simulink model "tg9"  (R2022a)
settings: Solver=ode15s  StartTime=0.0  StopTime=10  MaxStep=0.01  RelTol=1e-3
InitFcn:
  | mecha_param2
  | control_param0
values from neighbouring files (symbols this model uses):
  b0 = 0    [sim_IMMC.m]
  b1 = 1    [sim_IMMC.m]
  back0 = 0    [sim_IMMC.m]
  back1 = 0    [sim_IMMC.m]
  boff = 0    [sim_IMMC.m]
  bon = 0    [sim_IMMC.m]
  c = 0.05    [mecha_param2.m]
  c_jointstop = 0.3 / (pi/180)    (= 17.1887338539)    [mecha_param2.m]
  calctalus = sqrt((L_foot - (DJ1x_foot))^2 + (H_foot-r_cs)^2)    [mecha_param2.m]
  calctoes = sqrt((H_foot-r_cs)^2 + (DJ1x_foot)^2)    [mecha_param2.m]
  corrD = 0.001    [control_param0.m]
  DG_HAT = 0.35    [mecha_param2.m]
  DG_thigh = 0.28    [mecha_param2.m]
  DJ1x_foot = 0.16-r_cs    (= 0.135)    [mecha_param2.m]
  eref = 0.04    [mecha_param2.m]
  FmaxBFSH = 350    [mecha_param2.m]
  FmaxGAS = 1500    [mecha_param2.m]
  FmaxGLU = 1500    [mecha_param2.m]
  FmaxHAM = 3000    [mecha_param2.m]
  FmaxHFL = 2000    [mecha_param2.m]
  FmaxRF = 1200    [mecha_param2.m]
  FmaxSOL = 4000    [mecha_param2.m]
  FmaxTA = 800    [mecha_param2.m]
  FmaxVAS = 6000    [mecha_param2.m]
  g = 9.81    [mecha_param2.m]
  g0 = 0    [sim_IMMC.m]
  g1 = 0    [sim_IMMC.m]
  H_foot = 0.08    [mecha_param2.m]
  In_HAT = 3    [mecha_param2.m]
  In_shank = 0.05    [mecha_param2.m]
  In_thigh = 0.15    [mecha_param2.m]
  K = 5    [mecha_param2.m]
  knee_thigh = [0 0 -(L_thigh/2)]    [mecha_param2.m]
  Kpress = m_HAT * g / DeltaThRef    (= 104967)    [mecha_param2.m]
  L_foot = 0.2    [mecha_param2.m]
  L_HAT = 0.8    [mecha_param2.m]
  L_shank = 0.46    [mecha_param2.m]
  L_thigh = 0.46    [mecha_param2.m]
  LoHAM = table2array(mt('LoHAM', 1))    [control_param0.m]
  LoHFL = table2array(mt('LoHFL', 1))    [control_param0.m]
  longD = longD - corrD    (= 0.019)    [control_param0.m]
  loptBFSH = 0.12    [mecha_param2.m]
  loptGAS = 0.05    [mecha_param2.m]
  loptGLU = 0.11    [mecha_param2.m]
  loptHAM = 0.10    (= 0.1)    [mecha_param2.m]
  loptHFL = 0.11    [mecha_param2.m]
  loptRF = 0.08    [mecha_param2.m]
  loptSOL = 0.04    [mecha_param2.m]
  loptTA = 0.06    [mecha_param2.m]
  loptVAS = 0.08    [mecha_param2.m]
  LoTA = table2array(mt('LoTA', 1))    [control_param0.m]
  lslackBFSH = 0.10    (= 0.1)    [mecha_param2.m]
  lslackGAS = 0.40    (= 0.4)    [mecha_param2.m]
  lslackGLU = 0.13    [mecha_param2.m]
  lslackHAM = 0.31    [mecha_param2.m]
  lslackHFL = 0.10    (= 0.1)    [mecha_param2.m]
  lslackRF = 0.35    [mecha_param2.m]
  lslackSOL = 0.26    [mecha_param2.m]
  lslackTA = 0.24    [mecha_param2.m]
  lslackVAS = 0.23    [mecha_param2.m]
  m_HAT = 53.5    [mecha_param2.m]
  m_shank = 3.5    [mecha_param2.m]
  m_thigh = 8.5    [mecha_param2.m]
  midD = midD - corrD    (= 0.009)    [control_param0.m]
  N = 1.5    [mecha_param2.m]
  nonoff = 0    [control_param0.m]
  phi_a_low = (70) * (pi / 180)    (= 1.2217304764)    [mecha_param2.m]
  phi_a_up = (130) * (pi / 180)    (= 2.26892802759)    [mecha_param2.m]
  phi_dl = 180    [mecha_param2.m]
  phi_h = 230 * (pi / 180)    (= 4.01425727959)    [mecha_param2.m]
  phi_k = 175 * (pi / 180)    (= 3.05432619099)    [mecha_param2.m]
  phictoes = asind((DJ1y_foot-r_cs)/calctoes)    [mecha_param2.m]
  phimaxGASa = 100*pi/180    (= 1.74532925199)    [mecha_param2.m]
  phimaxGASk = 140*pi/180    (= 2.44346095279)    [mecha_param2.m]
  phimaxRFk = 165*pi/180    (= 2.87979326579)    [mecha_param2.m]
  phimaxSOL = 100*pi/180    (= 1.74532925199)    [mecha_param2.m]
  phimaxTA = 80*pi/180    (= 1.3962634016)    [mecha_param2.m]
  phimaxVAS = 165*pi/180    (= 2.87979326579)    [mecha_param2.m]
  phirefBFSH = 160*pi/180    (= 2.79252680319)    [mecha_param2.m]
  phirefGASa = 80*pi/180    (= 1.3962634016)    [mecha_param2.m]
  phirefGASk = 165*pi/180    (= 2.87979326579)    [mecha_param2.m]
  phirefGLU = 120*pi/180    (= 2.09439510239)    [mecha_param2.m]
  phirefHAMh = 150*pi/180    (= 2.61799387799)    [mecha_param2.m]
  phirefHAMk = 180*pi/180    (= 3.14159265359)    [mecha_param2.m]
  phirefHFL = 160*pi/180    (= 2.79252680319)    [mecha_param2.m]
  phirefRFh = 170*pi/180    (= 2.96705972839)    [mecha_param2.m]
  phirefRFk = 125*pi/180    (= 2.18166156499)    [mecha_param2.m]
  phirefSOL = 90*pi/180    (= 1.57079632679)    [mecha_param2.m]
  phirefTA = 110*pi/180    (= 1.91986217719)    [mecha_param2.m]
  phirefVAS = 120*pi/180    (= 2.09439510239)    [mecha_param2.m]
  phiScaleGASa = acos(rGASamin/rGASamax)/(phiminGASa-phimaxGASa)    [mecha_param2.m]
  phiScaleGASk = acos(rGASkmin/rGASkmax)/(phiminGASk-phimaxGASk)    [mecha_param2.m]
  phiScaleRFk = acos(rRFkmin/rRFkmax)/(phiminRFk-phimaxRFk)    [mecha_param2.m]
  phiScaleSOL = acos(rSOLmin/rSOLmax)/(phiminSOL-phimaxSOL)    [mecha_param2.m]
  phiScaleTA = acos(rTAmin/rTAmax)/(phiminTA-phimaxTA)    [mecha_param2.m]
  phiScaleVAS = acos(rVASmin/rVASmax)/(phiminVAS-phimaxVAS)    [mecha_param2.m]
  r1 = 0    [sim_IMMC.m]
  r_cs = 0.025    [mecha_param2.m]
  rBFSH = 0.04    [mecha_param2.m]
  rGASamax = 0.06    [mecha_param2.m]
  rGASkmax = 0.05    [mecha_param2.m]
  rGLU = 0.08    [mecha_param2.m]
  rHAMh = 0.08    [mecha_param2.m]
  rHAMk = 0.05    [mecha_param2.m]
  rHFL = 0.08    [mecha_param2.m]
  rhoBFSH = 0.7    [mecha_param2.m]
  rhoGASa = 0.7    [mecha_param2.m]
  rhoGASk = 0.7    [mecha_param2.m]
  rhoGLU = 0.5    [mecha_param2.m]
  rhoHAMh = 0.5    [mecha_param2.m]
  rhoHAMk = 0.5    [mecha_param2.m]
  rhoHFL = 0.5    [mecha_param2.m]
  rhoRFh = 0.3    [mecha_param2.m]
  rhoRFk = 0.5    [mecha_param2.m]
  rhoSOL = 0.5    [mecha_param2.m]
  rhoTA = 0.7    [mecha_param2.m]
  rhoVAS = 0.6    [mecha_param2.m]
  rRFh = 0.08    [mecha_param2.m]
  rRFkmax = 0.06    [mecha_param2.m]
  rSOLmax = 0.06    [mecha_param2.m]
  ... (+25 more)
undefined symbols (not defined in the file or in its folder): beta11, beta12, beta13, beta14, beta15, beta16, beta21, beta22, beta23, beta24, beta25, beta26, beta31, beta32, beta33, beta34, beta35, beta36, beta41, beta42, beta43, beta44, beta45, beta46, beta51, beta52, beta53, beta54, beta55, beta56, betab1, betab2, betab3, betab4, betab5, betab6, betap11, betap12, betap13, betap14, betap15, betap16, betap21, betap22, betap23, betap24, betap25, betap26, betap31, betap32, betap33, betap34, betap35, betap36, betap41, betap42, betap43, betap44, betap45, betap46 ... (+102)
libraries: sm_lib x89, simulink x72, nesl_utility x58, simulink_extras x18
(part 4 of 12)

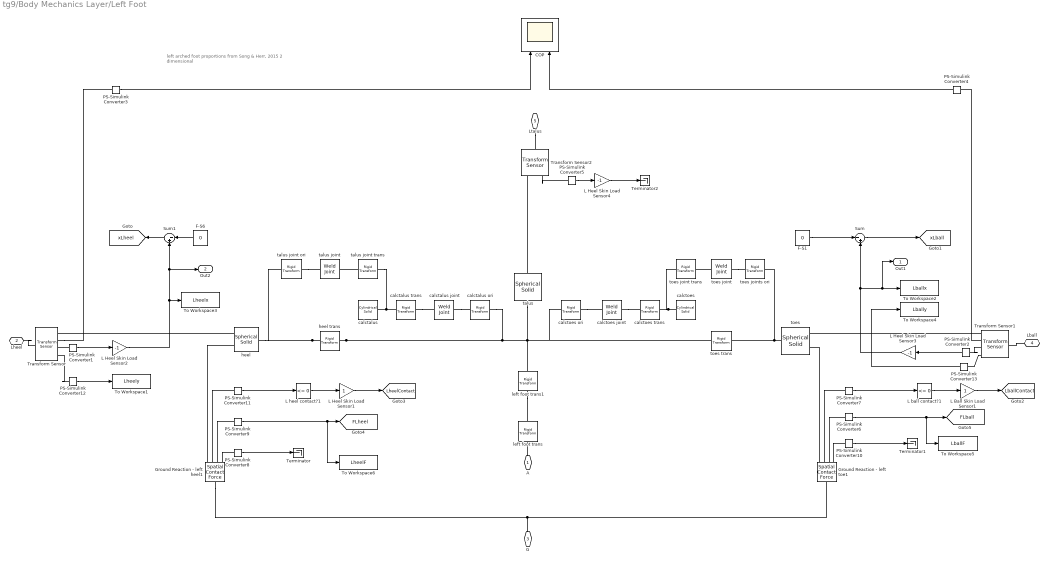
== system tg9/Body Mechanics Layer/Left Foot ==
  note: left arched foot
      | proportions from Song & Herr, 2015
      | 2 dimensional
  COP : Scope  NumInputPorts=2
  F-S1 : Constant  Value=0  OutDataTypeStr=Inherit: Inherit via back propagation
  F-S6 : Constant  Value=0  OutDataTypeStr=Inherit: Inherit via back propagation
  Ground Reaction - left heel1 : sm_lib/Forces and Torques/Spatial Contact Force  SenseContactBaseRotation=off  SenseContactBaseTranslation=off  CoefficientOfDynamicFriction=mu_static  CoefficientOfStaticFriction=mu_dynamic  NormalDamping=damp  NormalDampingUnits=N/(m/s)  SenseContactSignal=off  NormalStiffness=stiff  NormalStiffnessUnits=N/m  FrictionalCriticalVelocity=vLimit  FrictionalCriticalVelocityUnits=m/s  ZeroCrossDetectContactStartAndEnd=on  SenseContactFollowerRotation=off  SenseContactFollowerTranslation=off  FrictionType=SmoothStickSlip  SenseFrictionalForceMagnitude=on  SenseNormalForceMagnitude=on  NormalForceType=SmoothSpringDamper  SenseNormalVelocity=off  SenseSeparationDistance=on  SenseTangentialVelocity=off  NormalTransitionRegionWidth=trw  NormalTransitionRegionWidthUnits=m
  Ground Reaction - left toe1 : sm_lib/Forces and Torques/Spatial Contact Force  SenseContactBaseRotation=off  SenseContactBaseTranslation=off  CoefficientOfDynamicFriction=mu_static  CoefficientOfStaticFriction=mu_dynamic  NormalDamping=damp  NormalDampingUnits=N/(m/s)  SenseContactSignal=off  NormalStiffness=stiff  NormalStiffnessUnits=N/m  FrictionalCriticalVelocity=vLimit  FrictionalCriticalVelocityUnits=m/s  ZeroCrossDetectContactStartAndEnd=on  SenseContactFollowerRotation=off  SenseContactFollowerTranslation=off  FrictionType=SmoothStickSlip  SenseFrictionalForceMagnitude=on  SenseNormalForceMagnitude=on  NormalForceType=SmoothSpringDamper  SenseNormalVelocity=off  SenseSeparationDistance=on  SenseTangentialVelocity=off  NormalTransitionRegionWidth=trw  NormalTransitionRegionWidthUnits=m
  L Ball Skin Load Sensor1 : Gain
  L Heel Skin Load Sensor1 : Gain
  L Heel Skin Load Sensor2 : Gain  Gain=-1
  L Heel Skin Load Sensor3 : Gain  Gain=-1
  L Heel Skin Load Sensor4 : Gain  Gain=-1
  L ball contact?1 : simulink/Logic and Bit Operations/Compare To Zero  relop=<=  OutDataTypeStr=boolean
  L heel contact?1 : simulink/Logic and Bit Operations/Compare To Zero  relop=<=  OutDataTypeStr=boolean
  PS-Simulink Converter{1..13} (13 alike) : nesl_utility/PS-Simulink Converter  PhysicalDomain=network_engine_domain  SubClassName=ps_output  LeftPortType=input  RightPortType=output  PseudoPeriodic=off  Frequencies=[]  VectorFormat=1-D array  Unit=inherit  AffineConversion=off
      settings: SourceProductBaseCode=SS,PW,VE
  Sum : Sum  Inputs=|-+
  Sum1 : Sum  Inputs=|-+
  Terminator : Terminator
  Terminator1 : Terminator
  Terminator2 : Terminator
  To Workspace1 : ToWorkspace  VariableName=Lheely  SampleTime=-1
  To Workspace2 : ToWorkspace  VariableName=Lballx  SampleTime=-1
  To Workspace3 : ToWorkspace  VariableName=Lheelx  SampleTime=-1
  To Workspace4 : ToWorkspace  VariableName=Lbally  SampleTime=-1
  To Workspace5 : ToWorkspace  VariableName=LballF  SampleTime=-1
  To Workspace6 : ToWorkspace  VariableName=LheelF  SampleTime=-1
  Transform Sensor : sm_lib/Frames and Transforms/Transform Sensor  MeasurementFrame=World  SenseAngle=off  SenseAxis=off  SenseAngle1=off  SenseAngle2=off  SenseAngle3=off  SenseQ=off  SenseR=off  SenseOmegaX=off  SenseOmegaY=off  SenseOmegaZ=off  SenseOmega1=off  SenseOmega2=off  SenseOmega3=off  SenseQDot=off  SenseRDot=off  SenseAlphaX=off  SenseAlphaY=off  SenseAlphaZ=off  SenseAlpha1=off  SenseAlpha2=off  SenseAlpha3=off  SenseQDDot=off  SenseRDDot=off  SenseX=on  SenseY=on  SenseZ=on  SenseRad=off  SenseAzim=off  SenseDist=off  SenseInc=off  SenseXDot=off  SenseYDot=off  SenseZDot=off  SenseRadDot=off  SenseAzimDot=off  SenseDistDot=off  SenseIncDot=off  SenseXDDot=off  SenseYDDot=off  SenseZDDot=off  SenseRadDDot=off  SenseAzimDDot=off  SenseDistDDot=off  SenseIncDDot=off
  Transform Sensor1 : sm_lib/Frames and Transforms/Transform Sensor  MeasurementFrame=World  SenseAngle=off  SenseAxis=off  SenseAngle1=off  SenseAngle2=off  SenseAngle3=off  SenseQ=off  SenseR=off  SenseOmegaX=off  SenseOmegaY=off  SenseOmegaZ=off  SenseOmega1=off  SenseOmega2=off  SenseOmega3=off  SenseQDot=off  SenseRDot=off  SenseAlphaX=off  SenseAlphaY=off  SenseAlphaZ=off  SenseAlpha1=off  SenseAlpha2=off  SenseAlpha3=off  SenseQDDot=off  SenseRDDot=off  SenseX=on  SenseY=on  SenseZ=on  SenseRad=off  SenseAzim=off  SenseDist=off  SenseInc=off  SenseXDot=off  SenseYDot=off  SenseZDot=off  SenseRadDot=off  SenseAzimDot=off  SenseDistDot=off  SenseIncDot=off  SenseXDDot=off  SenseYDDot=off  SenseZDDot=off  SenseRadDDot=off  SenseAzimDDot=off  SenseDistDDot=off  SenseIncDDot=off
  Transform Sensor2 : sm_lib/Frames and Transforms/Transform Sensor  MeasurementFrame=World  SenseAngle=off  SenseAxis=off  SenseAngle1=off  SenseAngle2=off  SenseAngle3=off  SenseQ=off  SenseR=off  SenseOmegaX=off  SenseOmegaY=off  SenseOmegaZ=off  SenseOmega1=off  SenseOmega2=off  SenseOmega3=off  SenseQDot=off  SenseRDot=off  SenseAlphaX=off  SenseAlphaY=off  SenseAlphaZ=off  SenseAlpha1=off  SenseAlpha2=off  SenseAlpha3=off  SenseQDDot=off  SenseRDDot=off  SenseX=off  SenseY=on  SenseZ=off  SenseRad=off  SenseAzim=off  SenseDist=off  SenseInc=off  SenseXDot=off  SenseYDot=off  SenseZDot=off  SenseRadDot=off  SenseAzimDot=off  SenseDistDot=off  SenseIncDot=off  SenseXDDot=off  SenseYDDot=off  SenseZDDot=off  SenseRadDDot=off  SenseAzimDDot=off  SenseDistDDot=off  SenseIncDDot=off
  calctalus : sm_lib/Body Elements/Cylindrical Solid  GraphicAmbientColor=[0.15 0.15 0.15 1.0]  BasedOnType=Mass  CenterOfMass=[0 0 0]  CenterOfMassUnits=m  GraphicDiffuseColor=[0.5 0.5 0.5]  CylinderLength=calctalus  CylinderLengthUnits=m  CylinderRadius=0.02  CylinderRadiusUnits=m  Density=1000  DensityUnits=kg/m^3  DoExposeReferenceFrame=on  GraphicEmissiveColor=[0.0 0.0 0.0 1.0]  ExportEntireGeometry=off  SerializedFrames=<Frames/>  MarkerShape=Sphere  MarkerSize=10  GraphicType=FromGeometry  InertiaType=CalculateFromGeometry  Mass=0  MassUnits=kg  MomentsOfInertia=[1 1 1]  MomentsOfInertiaUnits=kg*m^2  GraphicOpacity=1.0  ProductsOfInertia=[0 0 0]  ProductsOfInertiaUnits=kg*m^2  GraphicShininess=75  GraphicSpecularColor=[0.5 0.5 0.5 1.0]  GraphicVisPropType=SimpleVisualProperties
  calctalus joint : sm_lib/Joints/Weld Joint  JointMode=Normal  SenseConstraintForce=off  SenseConstraintForceX=off  SenseConstraintForceY=off  SenseConstraintForceZ=off  SenseConstraintTorque=off  SenseConstraintTorqueX=off  SenseConstraintTorqueY=off  SenseConstraintTorqueZ=off  SenseTotalForce=off  SenseTotalForceX=off  SenseTotalForceY=off  SenseTotalForceZ=off  SenseTotalTorque=off  SenseTotalTorqueX=off  SenseTotalTorqueY=off  SenseTotalTorqueZ=off  CompositeWrenchDir=FollowerOnBase  CompositeWrenchFrame=BaseFrame
  calctalus ori : sm_lib/Frames and Transforms/Rigid Transform  TranslationMethod=None  TranslationStandardOffset=0  TranslationLengthUnit=m  TranslationStandardAxis=+Z  TranslationCartesianOffset=[0 0 -(calctoes/2)]  TranslationROffset=0  TranslationROffsetUnits=m  TranslationZOffset=0  TranslationZOffsetUnits=m  TranslationThetaOffset=0  TranslationThetaOffsetUnits=deg  RotationMethod=StandardAxis  RotationAngleUnits=deg  RotationStandardAxis=+Y  RotationAngle=phictalus  RotationArbitraryAxis=[0 0 1]  FollAlignAxisA=+X  BaseAlignAxisA=+Y  FollAlignAxisB=+Y  BaseAlignAxisB=+Z  RotationSequenceAxes=FollowerAxes  RotationSequence=XYX  RotationSequenceAngles=[0 0 0]  RotationSequenceAnglesUnits=deg  RotationMatrix=[1 0 0; 0 1 0; 0 0 1]
  calctalus trans : sm_lib/Frames and Transforms/Rigid Transform  TranslationMethod=Cartesian  TranslationStandardOffset=0  TranslationLengthUnit=m  TranslationStandardAxis=+Z  TranslationCartesianOffset=[0 0 -(calctalus/2)]  TranslationROffset=0  TranslationROffsetUnits=m  TranslationZOffset=0  TranslationZOffsetUnits=m  TranslationThetaOffset=0  TranslationThetaOffsetUnits=deg  RotationMethod=None  RotationAngleUnits=deg  RotationStandardAxis=+Y  RotationAngle=phictalus  RotationArbitraryAxis=[0 0 1]  FollAlignAxisA=+X  BaseAlignAxisA=+Y  FollAlignAxisB=+Y  BaseAlignAxisB=+Z  RotationSequenceAxes=FollowerAxes  RotationSequence=XYX  RotationSequenceAngles=[0 0 0]  RotationSequenceAnglesUnits=deg  RotationMatrix=[1 0 0; 0 1 0; 0 0 1]
  calctoes : sm_lib/Body Elements/Cylindrical Solid  GraphicAmbientColor=[0.15 0.15 0.15 1.0]  BasedOnType=Mass  CenterOfMass=[0 0 0]  CenterOfMassUnits=m  GraphicDiffuseColor=[0.5 0.5 0.5]  CylinderLength=calctoes  CylinderLengthUnits=m  CylinderRadius=0.02  CylinderRadiusUnits=m  Density=1000  DensityUnits=kg/m^3  DoExposeReferenceFrame=on  GraphicEmissiveColor=[0.0 0.0 0.0 1.0]  ExportEntireGeometry=off  SerializedFrames=<Frames/>  MarkerShape=Sphere  MarkerSize=10  GraphicType=FromGeometry  InertiaType=CalculateFromGeometry  Mass=0  MassUnits=kg  MomentsOfInertia=[1 1 1]  MomentsOfInertiaUnits=kg*m^2  GraphicOpacity=1.0  ProductsOfInertia=[0 0 0]  ProductsOfInertiaUnits=kg*m^2  GraphicShininess=75  GraphicSpecularColor=[0.5 0.5 0.5 1.0]  GraphicVisPropType=SimpleVisualProperties
  calctoes joint : sm_lib/Joints/Weld Joint  JointMode=Normal  SenseConstraintForce=off  SenseConstraintForceX=off  SenseConstraintForceY=off  SenseConstraintForceZ=off  SenseConstraintTorque=off  SenseConstraintTorqueX=off  SenseConstraintTorqueY=off  SenseConstraintTorqueZ=off  SenseTotalForce=off  SenseTotalForceX=off  SenseTotalForceY=off  SenseTotalForceZ=off  SenseTotalTorque=off  SenseTotalTorqueX=off  SenseTotalTorqueY=off  SenseTotalTorqueZ=off  CompositeWrenchDir=FollowerOnBase  CompositeWrenchFrame=BaseFrame
  calctoes ori : sm_lib/Frames and Transforms/Rigid Transform  TranslationMethod=None  TranslationStandardOffset=0  TranslationLengthUnit=m  TranslationStandardAxis=+Z  TranslationCartesianOffset=[0 0 -(calctoes/2)]  TranslationROffset=0  TranslationROffsetUnits=m  TranslationZOffset=0  TranslationZOffsetUnits=m  TranslationThetaOffset=0  TranslationThetaOffsetUnits=deg  RotationMethod=StandardAxis  RotationAngleUnits=deg  RotationStandardAxis=-Y  RotationAngle=90-phictoes  RotationArbitraryAxis=[0 0 1]  FollAlignAxisA=+X  BaseAlignAxisA=+Y  FollAlignAxisB=+Y  BaseAlignAxisB=+Z  RotationSequenceAxes=FollowerAxes  RotationSequence=XYX  RotationSequenceAngles=[0 0 0]  RotationSequenceAnglesUnits=deg  RotationMatrix=[1 0 0; 0 1 0; 0 0 1]
  calctoes trans : sm_lib/Frames and Transforms/Rigid Transform  TranslationMethod=Cartesian  TranslationStandardOffset=0  TranslationLengthUnit=m  TranslationStandardAxis=+Z  TranslationCartesianOffset=[0 0 -(calctoes/2)]  TranslationROffset=0  TranslationROffsetUnits=m  TranslationZOffset=0  TranslationZOffsetUnits=m  TranslationThetaOffset=0  TranslationThetaOffsetUnits=deg  RotationMethod=None  RotationAngleUnits=deg  RotationStandardAxis=-Y  RotationAngle=90-phictoes  RotationArbitraryAxis=[0 0 1]  FollAlignAxisA=+X  BaseAlignAxisA=+Y  FollAlignAxisB=+Y  BaseAlignAxisB=+Z  RotationSequenceAxes=FollowerAxes  RotationSequence=XYX  RotationSequenceAngles=[0 0 0]  RotationSequenceAnglesUnits=deg  RotationMatrix=[1 0 0; 0 1 0; 0 0 1]
  heel : sm_lib/Body Elements/Spherical Solid  GraphicAmbientColor=[0.15 0.15 0.15 1.0]  BasedOnType=Mass  CenterOfMass=[0 0 0]  CenterOfMassUnits=m  GraphicDiffuseColor=[1.0 0.0 0.2]  Density=1000  DensityUnits=kg/m^3  DoExposeReferenceFrame=on  GraphicEmissiveColor=[0.0 0.0 0.0 1.0]  ExportEntireGeometry=on  SerializedExposedGeometries=<ExposedGeometries/>  SerializedFrames=<Frames><Frame><Id>Frame1</Id><Value><Name>COM</Name><Origin><Source>CenterOfMassFrame</Source><FeatureName></FeatureName></Origin><PrimaryAxis><DefinedDirection>+Z</DefinedDirection><Source>ReferenceFrame</Source><SourceDirection>+Z</SourceDirection><FeatureName></FeatureName></PrimaryAxis><SecondaryAxis><DefinedDirection>+X</DefinedDirection><Source>ReferenceFrame</Source><SourceDirection>+X</SourceDirection><FeatureName></FeatureName></SecondaryAxis></Value></Frame></Frames>  MarkerShape=Sphere  MarkerSize=10  GraphicType=FromGeometry  InertiaType=CalculateFromGeometry  Mass=0  MassUnits=kg  MomentsOfInertia=[1 1 1]  MomentsOfInertiaUnits=kg*m^2  GraphicOpacity=1.0  ProductsOfInertia=[0 0 0]  ProductsOfInertiaUnits=kg*m^2  GraphicShininess=75  GraphicSpecularColor=[0.5 0.5 0.5 1.0]  SphereRadius=r_cs  SphereRadiusUnits=m  GraphicVisPropType=SimpleVisualProperties
  heel trans : sm_lib/Frames and Transforms/Rigid Transform  TranslationMethod=Cartesian  TranslationStandardOffset=0  TranslationLengthUnit=m  TranslationStandardAxis=+Z  TranslationCartesianOffset=[(DJ1x_foot - L_foot) 0 (r_cs-H_foot)]  TranslationROffset=0  TranslationROffsetUnits=m  TranslationZOffset=0  TranslationZOffsetUnits=m  TranslationThetaOffset=0  TranslationThetaOffsetUnits=deg  RotationMethod=None  RotationAngleUnits=deg  RotationStandardAxis=+Y  RotationAngle=phictalus  RotationArbitraryAxis=[0 0 1]  FollAlignAxisA=+X  BaseAlignAxisA=+Y  FollAlignAxisB=+Y  BaseAlignAxisB=+Z  RotationSequenceAxes=FollowerAxes  RotationSequence=XYX  RotationSequenceAngles=[0 0 0]  RotationSequenceAnglesUnits=deg  RotationMatrix=[1 0 0; 0 1 0; 0 0 1]
  left foot trans : sm_lib/Frames and Transforms/Rigid Transform  TranslationMethod=None  TranslationStandardOffset=0  TranslationLengthUnit=m  TranslationStandardAxis=+Z  TranslationCartesianOffset=[]  TranslationROffset=0  TranslationROffsetUnits=m  TranslationZOffset=0  TranslationZOffsetUnits=m  TranslationThetaOffset=0  TranslationThetaOffsetUnits=deg  RotationMethod=StandardAxis  RotationAngleUnits=deg  RotationStandardAxis=+Y  RotationAngle=90  RotationArbitraryAxis=[0 0 1]  FollAlignAxisA=+X  BaseAlignAxisA=+Y  FollAlignAxisB=+Y  BaseAlignAxisB=+Z  RotationSequenceAxes=FollowerAxes  RotationSequence=XYX  RotationSequenceAngles=[0 0 0]  RotationSequenceAnglesUnits=deg  RotationMatrix=[1 0 0; 0 1 0; 0 0 1]
  left foot trans1 : sm_lib/Frames and Transforms/Rigid Transform  TranslationMethod=None  TranslationStandardOffset=0  TranslationLengthUnit=m  TranslationStandardAxis=+Z  TranslationCartesianOffset=[]  TranslationROffset=0  TranslationROffsetUnits=m  TranslationZOffset=0  TranslationZOffsetUnits=m  TranslationThetaOffset=0  TranslationThetaOffsetUnits=deg  RotationMethod=StandardAxis  RotationAngleUnits=deg  RotationStandardAxis=-Z  RotationAngle=90  RotationArbitraryAxis=[0 0 1]  FollAlignAxisA=+X  BaseAlignAxisA=+Y  FollAlignAxisB=+Y  BaseAlignAxisB=+Z  RotationSequenceAxes=FollowerAxes  RotationSequence=XYX  RotationSequenceAngles=[0 0 0]  RotationSequenceAnglesUnits=deg  RotationMatrix=[1 0 0; 0 1 0; 0 0 1]
  talus : sm_lib/Body Elements/Spherical Solid  GraphicAmbientColor=[0.15 0.15 0.15 1.0]  BasedOnType=Density  CenterOfMass=cm_foot  CenterOfMassUnits=m  GraphicDiffuseColor=[0.6 1.0 1.0]  Density=1000  DensityUnits=kg/m^3  DoExposeReferenceFrame=on  GraphicEmissiveColor=[0.0 0.0 0.0 1.0]  ExportEntireGeometry=off  SerializedExposedGeometries=<ExposedGeometries/>  SerializedFrames=<Frames><Frame><Id>Frame1</Id><Value><Name>COM</Name><Origin><Source>ReferenceFrame</Source><FeatureName></FeatureName></Origin><PrimaryAxis><DefinedDirection>+Z</DefinedDirection><Source>ReferenceFrame</Source><SourceDirection>+Z</SourceDirection><FeatureName></FeatureName></PrimaryAxis><SecondaryAxis><DefinedDirection>+X</DefinedDirection><Source>ReferenceFrame</Source><SourceDirection>+X</SourceDirection><FeatureName></FeatureName></SecondaryAxis></Value></Frame></Frames>  MarkerShape=Sphere  MarkerSize=10  GraphicType=FromGeometry  InertiaType=Custom  Mass=1.25  MassUnits=kg  MomentsOfInertia=[0 0.005 0]  MomentsOfInertiaUnits=kg*m^2  GraphicOpacity=1.0  ProductsOfInertia=[0 0 0]  ProductsOfInertiaUnits=kg*m^2  GraphicShininess=75  GraphicSpecularColor=[0.5 0.5 0.5 1.0]  SphereRadius=r_foot  SphereRadiusUnits=m  GraphicVisPropType=SimpleVisualProperties
  talus joint : sm_lib/Joints/Weld Joint  JointMode=Normal  SenseConstraintForce=off  SenseConstraintForceX=off  SenseConstraintForceY=off  SenseConstraintForceZ=off  SenseConstraintTorque=off  SenseConstraintTorqueX=off  SenseConstraintTorqueY=off  SenseConstraintTorqueZ=off  SenseTotalForce=off  SenseTotalForceX=off  SenseTotalForceY=off  SenseTotalForceZ=off  SenseTotalTorque=off  SenseTotalTorqueX=off  SenseTotalTorqueY=off  SenseTotalTorqueZ=off  CompositeWrenchDir=FollowerOnBase  CompositeWrenchFrame=BaseFrame
  talus joint ori : sm_lib/Frames and Transforms/Rigid Transform  TranslationMethod=None  TranslationStandardOffset=0  TranslationLengthUnit=m  TranslationStandardAxis=+Z  TranslationCartesianOffset=[0 0 -(calctoes/2)]  TranslationROffset=0  TranslationROffsetUnits=m  TranslationZOffset=0  TranslationZOffsetUnits=m  TranslationThetaOffset=0  TranslationThetaOffsetUnits=deg  RotationMethod=StandardAxis  RotationAngleUnits=deg  RotationStandardAxis=-Y  RotationAngle=phictalus  RotationArbitraryAxis=[0 0 1]  FollAlignAxisA=+X  BaseAlignAxisA=+Y  FollAlignAxisB=+Y  BaseAlignAxisB=+Z  RotationSequenceAxes=FollowerAxes  RotationSequence=XYX  RotationSequenceAngles=[0 0 0]  RotationSequenceAnglesUnits=deg  RotationMatrix=[1 0 0; 0 1 0; 0 0 1]
  talus joint trans : sm_lib/Frames and Transforms/Rigid Transform  TranslationMethod=Cartesian  TranslationStandardOffset=0  TranslationLengthUnit=m  TranslationStandardAxis=+Z  TranslationCartesianOffset=[0 0 -(calctalus/2)]  TranslationROffset=0  TranslationROffsetUnits=m  TranslationZOffset=0  TranslationZOffsetUnits=m  TranslationThetaOffset=0  TranslationThetaOffsetUnits=deg  RotationMethod=None  RotationAngleUnits=deg  RotationStandardAxis=+Y  RotationAngle=phictalus  RotationArbitraryAxis=[0 0 1]  FollAlignAxisA=+X  BaseAlignAxisA=+Y  FollAlignAxisB=+Y  BaseAlignAxisB=+Z  RotationSequenceAxes=FollowerAxes  RotationSequence=XYX  RotationSequenceAngles=[0 0 0]  RotationSequenceAnglesUnits=deg  RotationMatrix=[1 0 0; 0 1 0; 0 0 1]
  toes : sm_lib/Body Elements/Spherical Solid  GraphicAmbientColor=[0.15 0.15 0.15 1.0]  BasedOnType=Mass  CenterOfMass=[0 0 0]  CenterOfMassUnits=m  GraphicDiffuseColor=[1.0 0.0 0.2]  Density=1000  DensityUnits=kg/m^3  DoExposeReferenceFrame=on  GraphicEmissiveColor=[0.0 0.0 0.0 1.0]  ExportEntireGeometry=on  SerializedExposedGeometries=<ExposedGeometries/>  SerializedFrames=<Frames><Frame><Id>Frame1</Id><Value><Name>COM</Name><Origin><Source>CenterOfMassFrame</Source><FeatureName></FeatureName></Origin><PrimaryAxis><DefinedDirection>+Z</DefinedDirection><Source>ReferenceFrame</Source><SourceDirection>+Z</SourceDirection><FeatureName></FeatureName></PrimaryAxis><SecondaryAxis><DefinedDirection>+X</DefinedDirection><Source>ReferenceFrame</Source><SourceDirection>+X</SourceDirection><FeatureName></FeatureName></SecondaryAxis></Value></Frame></Frames>  MarkerShape=Sphere  MarkerSize=10  GraphicType=FromGeometry  InertiaType=CalculateFromGeometry  Mass=0  MassUnits=kg  MomentsOfInertia=[1 1 1]  MomentsOfInertiaUnits=kg*m^2  GraphicOpacity=1.0  ProductsOfInertia=[0 0 0]  ProductsOfInertiaUnits=kg*m^2  GraphicShininess=75  GraphicSpecularColor=[0.5 0.5 0.5 1.0]  SphereRadius=r_cs  SphereRadiusUnits=m  GraphicVisPropType=SimpleVisualProperties
  toes joint : sm_lib/Joints/Weld Joint  JointMode=Normal  SenseConstraintForce=off  SenseConstraintForceX=off  SenseConstraintForceY=off  SenseConstraintForceZ=off  SenseConstraintTorque=off  SenseConstraintTorqueX=off  SenseConstraintTorqueY=off  SenseConstraintTorqueZ=off  SenseTotalForce=off  SenseTotalForceX=off  SenseTotalForceY=off  SenseTotalForceZ=off  SenseTotalTorque=off  SenseTotalTorqueX=off  SenseTotalTorqueY=off  SenseTotalTorqueZ=off  CompositeWrenchDir=FollowerOnBase  CompositeWrenchFrame=BaseFrame
  toes joint trans : sm_lib/Frames and Transforms/Rigid Transform  TranslationMethod=Cartesian  TranslationStandardOffset=0  TranslationLengthUnit=m  TranslationStandardAxis=+Z  TranslationCartesianOffset=[0 0 -(calctoes/2)]  TranslationROffset=0  TranslationROffsetUnits=m  TranslationZOffset=0  TranslationZOffsetUnits=m  TranslationThetaOffset=0  TranslationThetaOffsetUnits=deg  RotationMethod=None  RotationAngleUnits=deg  RotationStandardAxis=-Y  RotationAngle=90-phictoes  RotationArbitraryAxis=[0 0 1]  FollAlignAxisA=+X  BaseAlignAxisA=+Y  FollAlignAxisB=+Y  BaseAlignAxisB=+Z  RotationSequenceAxes=FollowerAxes  RotationSequence=XYX  RotationSequenceAngles=[0 0 0]  RotationSequenceAnglesUnits=deg  RotationMatrix=[1 0 0; 0 1 0; 0 0 1]
  toes joints ori : sm_lib/Frames and Transforms/Rigid Transform  TranslationMethod=None  TranslationStandardOffset=0  TranslationLengthUnit=m  TranslationStandardAxis=+Z  TranslationCartesianOffset=[0 0 -(calctoes/2)]  TranslationROffset=0  TranslationROffsetUnits=m  TranslationZOffset=0  TranslationZOffsetUnits=m  TranslationThetaOffset=0  TranslationThetaOffsetUnits=deg  RotationMethod=StandardAxis  RotationAngleUnits=deg  RotationStandardAxis=+Y  RotationAngle=90-phictoes  RotationArbitraryAxis=[0 0 1]  FollAlignAxisA=+X  BaseAlignAxisA=+Y  FollAlignAxisB=+Y  BaseAlignAxisB=+Z  RotationSequenceAxes=FollowerAxes  RotationSequence=XYX  RotationSequenceAngles=[0 0 0]  RotationSequenceAnglesUnits=deg  RotationMatrix=[1 0 0; 0 1 0; 0 0 1]
  toes trans : sm_lib/Frames and Transforms/Rigid Transform  TranslationMethod=Cartesian  TranslationStandardOffset=0  TranslationLengthUnit=m  TranslationStandardAxis=+Z  TranslationCartesianOffset=[(DJ1x_foot ) 0 (r_cs-H_foot)]  TranslationROffset=0  TranslationROffsetUnits=m  TranslationZOffset=0  TranslationZOffsetUnits=m  TranslationThetaOffset=0  TranslationThetaOffsetUnits=deg  RotationMethod=None  RotationAngleUnits=deg  RotationStandardAxis=-Y  RotationAngle=90-phictoes  RotationArbitraryAxis=[0 0 1]  FollAlignAxisA=+X  BaseAlignAxisA=+Y  FollAlignAxisB=+Y  BaseAlignAxisB=+Z  RotationSequenceAxes=FollowerAxes  RotationSequence=XYX  RotationSequenceAngles=[0 0 0]  RotationSequenceAnglesUnits=deg  RotationMatrix=[1 0 0; 0 1 0; 0 0 1]
  A : PMIOPort  Side=Left
  Lheel : PMIOPort  Port=2  Side=Left
  G : PMIOPort  Port=3  Side=Right
  Lball : PMIOPort  Port=4  Side=Left
  Ltalus : PMIOPort  Port=5  Side=Left
  Out1 : Outport
  Out2 : Outport  Port=2
  tag scope: FLball=global, FLheel=global, LballContact=global, LheelContact=global, xLball=global, xLheel=global
  wires:
  PS-Simulink Converter8/1 -> Terminator/1
  PS-Simulink Converter9/1 -> To Workspace6/1, [FLheel]
  PS-Simulink Converter11/1 -> L heel contact?1/1
  L ball contact?1/1 -> L Ball Skin Load Sensor1/1
  L Ball Skin Load Sensor1/1 -> [LballContact]
  L heel contact?1/1 -> L Heel Skin Load Sensor1/1
  L Heel Skin Load Sensor1/1 -> [LheelContact]
  PS-Simulink Converter7/1 -> L ball contact?1/1
  PS-Simulink Converter6/1 -> To Workspace5/1, [FLball]
  PS-Simulink Converter10/1 -> Terminator1/1
  PS-Simulink Converter2/1 -> L Heel Skin Load Sensor3/1
  PS-Simulink Converter1/1 -> L Heel Skin Load Sensor2/1
  L Heel Skin Load Sensor2/1 -> To Workspace3/1, Out2/1, Sum1/2
  L Heel Skin Load Sensor3/1 -> Out1/1, To Workspace2/1, Sum/2
  PS-Simulink Converter4/1 -> COP/2
  PS-Simulink Converter3/1 -> COP/1
  PS-Simulink Converter5/1 -> L Heel Skin Load Sensor4/1
  Sum/1 -> [xLball]
  Sum1/1 -> [xLheel]
  F-S6/1 -> Sum1/1
  F-S1/1 -> Sum/1
  L Heel Skin Load Sensor4/1 -> Terminator2/1
  PS-Simulink Converter12/1 -> To Workspace1/1
  PS-Simulink Converter13/1 -> To Workspace4/1
  connections:
  A/RConn1 -- left foot trans/LConn1
  Ground Reaction - left heel1/LConn1 -- Ground Reaction - left toe1/LConn1 -- G/RConn1
  heel trans/RConn1 -- heel/RConn1 -- talus joint ori/RConn1
  heel trans/LConn1 -- calctalus ori/LConn1 -- calctoes ori/LConn1 -- toes trans/LConn1 -- talus/RConn1 -- left foot trans1/RConn1
  calctalus trans/RConn1 -- talus joint trans/LConn1 -- calctalus/RConn1
  toes/RConn1 -- toes joints ori/RConn1 -- toes trans/RConn1
  calctoes/RConn1 -- toes joint trans/LConn1 -- calctoes trans/RConn1
  Ground Reaction - left toe1/RConn3 -- PS-Simulink Converter6/LConn1
  PS-Simulink Converter11/LConn1 -- Ground Reaction - left heel1/RConn2
  calctalus trans/LConn1 -- calctalus joint/RConn1
  calctalus joint/LConn1 -- calctalus ori/RConn1
  toes joint/LConn1 -- toes joint trans/RConn1
  talus joint ori/LConn1 -- talus joint/RConn1
  Ground Reaction - left heel1/RConn3 -- PS-Simulink Converter9/LConn1
  talus joint trans/RConn1 -- talus joint/LConn1
  PS-Simulink Converter8/LConn1 -- Ground Reaction - left heel1/RConn4
  toes joint/RConn1 -- toes joints ori/LConn1
  calctoes ori/RConn1 -- calctoes joint/LConn1
  Ground Reaction - left toe1/RConn1 -- toes/LConn2
  Ground Reaction - left toe1/RConn2 -- PS-Simulink Converter7/LConn1
  calctoes joint/RConn1 -- calctoes trans/LConn1
  Ground Reaction - left toe1/RConn4 -- PS-Simulink Converter10/LConn1
  left foot trans1/LConn1 -- left foot trans/RConn1
  heel/LConn2 -- Ground Reaction - left heel1/RConn1
  heel/LConn1 -- Transform Sensor/RConn1
  Lheel/RConn1 -- Transform Sensor/LConn1
  PS-Simulink Converter1/LConn1 -- Transform Sensor/RConn3
  Transform Sensor1/RConn1 -- toes/LConn1
  Lball/RConn1 -- Transform Sensor1/LConn1
  PS-Simulink Converter2/LConn1 -- Transform Sensor1/RConn3
  Transform Sensor/RConn2 -- PS-Simulink Converter3/LConn1
  Transform Sensor1/RConn2 -- PS-Simulink Converter4/LConn1
  Ltalus/RConn1 -- Transform Sensor2/LConn1
  Transform Sensor2/RConn2 -- PS-Simulink Converter5/LConn1
  talus/LConn1 -- Transform Sensor2/RConn1
  PS-Simulink Converter12/LConn1 -- Transform Sensor/RConn4
  PS-Simulink Converter13/LConn1 -- Transform Sensor1/RConn4

== system tg9/Body Mechanics Layer/Left Leg ==
  note: Left Leg - Mechanic Layer
  Gain{,1..3} (4 alike) : Gain  Gain=-1
  Gain4 : Gain
  L Knee Joint Sensor : Gain
  L Thigh Displacement Sensor : Gain
  Left Ankle : sm_lib/Joints/Revolute Joint  JointMode=Normal  SenseConstraintForce=off  SenseConstraintForceX=off  SenseConstraintForceY=off  SenseConstraintForceZ=off  SenseConstraintTorque=off  SenseConstraintTorqueX=off  SenseConstraintTorqueY=off  SenseConstraintTorqueZ=off  SenseTotalForce=off  SenseTotalForceX=off  SenseTotalForceY=off  SenseTotalForceZ=off  SenseTotalTorque=off  SenseTotalTorqueX=off  SenseTotalTorqueY=off  SenseTotalTorqueZ=off  CompositeWrenchDir=FollowerOnBase  CompositeWrenchFrame=BaseFrame  EquilibriumPosition=0  EquilibriumPositionUnits=deg  SpringStiffness=0  SpringStiffnessUnits=N*m/deg  DampingCoefficient=0  DampingCoefficientUnits=N*m/(deg/s)  TorqueActuationMode=InputTorque  MotionActuationMode=ComputedMotion  SensePosition=on  SenseVelocity=on  SenseAcceleration=off  SenseTorqueForce=off  SenseLowerLimitTorqueForce=off  SenseUpperLimitTorqueForce=off  LowerLimitSpecify=off  LowerLimitBound=-phi_dl  LowerLimitBoundUnits=deg  LowerLimitStiffness=1e4  LowerLimitStiffnessUnits=N*m/deg  LowerLimitDamping=10  LowerLimitDampingUnits=N*m/(deg/s)  LowerLimitTransitionRegionWidth=0.1  LowerLimitTransitionRegionWidthUnits=deg  UpperLimitSpecify=off  UpperLimitBound=phi_dl  UpperLimitBoundUnits=deg  UpperLimitStiffness=1e4  UpperLimitStiffnessUnits=N*m/deg  UpperLimitDamping=10  UpperLimitDampingUnits=N*m/(deg/s)  UpperLimitTransitionRegionWidth=0.1  UpperLimitTransitionRegionWidthUnits=deg  PositionTargetSpecify=on  PositionTargetPriority=High  PositionTargetValue=0  PositionTargetValueUnits=deg  VelocityTargetSpecify=off  VelocityTargetPriority=High  VelocityTargetValue=0  VelocityTargetValueUnits=deg/s
  Left Hip : sm_lib/Joints/Revolute Joint  JointMode=Normal  SenseConstraintForce=off  SenseConstraintForceX=off  SenseConstraintForceY=off  SenseConstraintForceZ=off  SenseConstraintTorque=off  SenseConstraintTorqueX=off  SenseConstraintTorqueY=off  SenseConstraintTorqueZ=off  SenseTotalForce=off  SenseTotalForceX=off  SenseTotalForceY=off  SenseTotalForceZ=off  SenseTotalTorque=off  SenseTotalTorqueX=off  SenseTotalTorqueY=off  SenseTotalTorqueZ=off  CompositeWrenchDir=FollowerOnBase  CompositeWrenchFrame=BaseFrame  EquilibriumPosition=0  EquilibriumPositionUnits=deg  SpringStiffness=0  SpringStiffnessUnits=N*m/deg  DampingCoefficient=0  DampingCoefficientUnits=N*m/(deg/s)  TorqueActuationMode=InputTorque  MotionActuationMode=ComputedMotion  SensePosition=on  SenseVelocity=on  SenseAcceleration=off  SenseTorqueForce=off  SenseLowerLimitTorqueForce=off  SenseUpperLimitTorqueForce=off  LowerLimitSpecify=off  LowerLimitBound=-phi_dl  LowerLimitBoundUnits=deg  LowerLimitStiffness=1e4  LowerLimitStiffnessUnits=N*m/deg  LowerLimitDamping=10  LowerLimitDampingUnits=N*m/(deg/s)  LowerLimitTransitionRegionWidth=0.1  LowerLimitTransitionRegionWidthUnits=deg  UpperLimitSpecify=off  UpperLimitBound=phi_dl  UpperLimitBoundUnits=deg  UpperLimitStiffness=1e4  UpperLimitStiffnessUnits=N*m/deg  UpperLimitDamping=10  UpperLimitDampingUnits=N*m/(deg/s)  UpperLimitTransitionRegionWidth=0.1  UpperLimitTransitionRegionWidthUnits=deg  PositionTargetSpecify=on  PositionTargetPriority=High  PositionTargetValue=0  PositionTargetValueUnits=rad  VelocityTargetSpecify=off  VelocityTargetPriority=High  VelocityTargetValue=0  VelocityTargetValueUnits=deg/s
  Left Knee : sm_lib/Joints/Revolute Joint  JointMode=Normal  SenseConstraintForce=off  SenseConstraintForceX=off  SenseConstraintForceY=off  SenseConstraintForceZ=off  SenseConstraintTorque=off  SenseConstraintTorqueX=off  SenseConstraintTorqueY=off  SenseConstraintTorqueZ=off  SenseTotalForce=off  SenseTotalForceX=off  SenseTotalForceY=off  SenseTotalForceZ=off  SenseTotalTorque=off  SenseTotalTorqueX=off  SenseTotalTorqueY=off  SenseTotalTorqueZ=off  CompositeWrenchDir=FollowerOnBase  CompositeWrenchFrame=BaseFrame  EquilibriumPosition=0  EquilibriumPositionUnits=deg  SpringStiffness=0  SpringStiffnessUnits=N*m/deg  DampingCoefficient=0  DampingCoefficientUnits=N*m/(deg/s)  TorqueActuationMode=InputTorque  MotionActuationMode=ComputedMotion  SensePosition=on  SenseVelocity=on  SenseAcceleration=off  SenseTorqueForce=off  SenseLowerLimitTorqueForce=off  SenseUpperLimitTorqueForce=off  LowerLimitSpecify=off  LowerLimitBound=-phi_dl  LowerLimitBoundUnits=deg  LowerLimitStiffness=1e4  LowerLimitStiffnessUnits=N*m/deg  LowerLimitDamping=10  LowerLimitDampingUnits=N*m/(deg/s)  LowerLimitTransitionRegionWidth=0.1  LowerLimitTransitionRegionWidthUnits=deg  UpperLimitSpecify=off  UpperLimitBound=phi_dl  UpperLimitBoundUnits=deg  UpperLimitStiffness=1e4  UpperLimitStiffnessUnits=N*m/deg  UpperLimitDamping=10  UpperLimitDampingUnits=N*m/(deg/s)  UpperLimitTransitionRegionWidth=0.1  UpperLimitTransitionRegionWidthUnits=deg  PositionTargetSpecify=on  PositionTargetPriority=High  PositionTargetValue=0  PositionTargetValueUnits=rad  VelocityTargetSpecify=off  VelocityTargetPriority=High  VelocityTargetValue=0  VelocityTargetValueUnits=deg/s
  Left Shank : sm_lib/Body Elements/Cylindrical Solid  GraphicAmbientColor=[0.15 0.15 0.15 1.0]  BasedOnType=Density  CenterOfMass=[0 0 -((L_shank/2)-DG_thigh)]  CenterOfMassUnits=m  GraphicDiffuseColor=bcolor  CylinderLength=L_shank  CylinderLengthUnits=m  CylinderRadius=r_shank  CylinderRadiusUnits=m  Density=1000  DensityUnits=kg/m^3  DoExposeReferenceFrame=on  GraphicEmissiveColor=[0.0 0.0 0.0 1.0]  ExportEntireGeometry=off  SerializedFrames=<Frames/>  MarkerShape=Sphere  MarkerSize=10  GraphicType=FromGeometry  InertiaType=Custom  Mass=m_shank  MassUnits=kg  MomentsOfInertia=[1 0 0]*In_shank  MomentsOfInertiaUnits=kg*m^2  GraphicOpacity=1.0  ProductsOfInertia=[0 0 0]  ProductsOfInertiaUnits=kg*m^2  GraphicShininess=75  GraphicSpecularColor=[0.5 0.5 0.5 1.0]  GraphicVisPropType=SimpleVisualProperties
  Left Thigh : Subsystem
      settings: PortSchema="{\"entries\":[{\"content\":{\"sides\":[{\"content\":{\"connectorIds\":[\"LConn1\"]},\"type\":\"ConnectorPlacement.EquallySpacedRectSide\",\"uuid\":\"691415be-cb86-489e-bec2-766d63ddca41\"},{\"content\":{\"connectorIds\":[\"RConn1\"],\"side\":\"RIGHT\"},\"type\":\"ConnectorPlacement.EquallySpacedRectSide\",\"uuid\":\"3de97b41-0b4c-4761-bb81-ab1a0e227fe0\"},{\"content\":{\"connectorIds\":[\"Out1\"],\"side\":\"TOP\"},\"type\":\"ConnectorPlacement.EquallySpacedRectSide\",\"uuid\":\"7408afde-6568-4d46-a226-b68b5f0b0811\"}]},\"type\":\"ConnectorPlacement.EquallySpacedConnector\",\"uuid\":\"10d26049-9991-4eaa-9e92-afa7abdb8957\"}],\"packageUris\":[\"http://schema.mathworks.com/mf0/Connector/R2020b\"],\"version\":\"1.0\"}"
  Left hip trans : sm_lib/Frames and Transforms/Rigid Transform  TranslationMethod=Cartesian  TranslationStandardOffset=0  TranslationLengthUnit=m  TranslationStandardAxis=+Z  TranslationCartesianOffset=hipL_HAT  TranslationROffset=0  TranslationROffsetUnits=m  TranslationZOffset=0  TranslationZOffsetUnits=m  TranslationThetaOffset=0  TranslationThetaOffsetUnits=deg  RotationMethod=StandardAxis  RotationAngleUnits=deg  RotationStandardAxis=+Y  RotationAngle=-90  RotationArbitraryAxis=[0 0 1]  FollAlignAxisA=+X  BaseAlignAxisA=+Y  FollAlignAxisB=+Y  BaseAlignAxisB=+Z  RotationSequenceAxes=FollowerAxes  RotationSequence=XYX  RotationSequenceAngles=[0 0 0]  RotationSequenceAnglesUnits=deg  RotationMatrix=[1 0 0; 0 1 0; 0 0 1]
  Mux{,1..3} (4 alike) : Mux  Inputs=2
  PS-Simulink Converter{,1,3..5} (5 alike) : nesl_utility/PS-Simulink Converter  PhysicalDomain=network_engine_domain  SubClassName=ps_output  LeftPortType=input  RightPortType=output  PseudoPeriodic=off  Frequencies=[]  VectorFormat=1-D array  Unit=inherit  AffineConversion=off
      settings: SourceProductBaseCode=SS,PW,VE
  PS-Simulink Converter2 : nesl_utility/PS-Simulink Converter  PhysicalDomain=network_engine_domain  SubClassName=ps_output  LeftPortType=input  RightPortType=output  PseudoPeriodic=off  Frequencies=[]  VectorFormat=1-D array  Unit=rad  AffineConversion=off
      settings: SourceProductBaseCode=SS,PW,VE
  Simulink-PS Converter : nesl_utility/Simulink-PS Converter  PhysicalDomain=network_engine_domain  SubClassName=ps_input  LeftPortType=input  RightPortType=output  PseudoPeriodic=off  Frequencies=[]  NoiseDistribution=none  NoiseParameters=[]  Unit=1  AffineConversion=off  FilteringAndDerivatives=provide  SimscapeFilterOrder=1  InputFilterTimeConstant=0.001  UdotUserProvided=0
      settings: SourceProductBaseCode=SS,PW,VE
  Simulink-PS Converter1 : nesl_utility/Simulink-PS Converter  PhysicalDomain=network_engine_domain  SubClassName=ps_input  LeftPortType=input  RightPortType=output  PseudoPeriodic=off  Frequencies=[]  NoiseDistribution=none  NoiseParameters=[]  Unit=1  AffineConversion=off  FilteringAndDerivatives=provide  SimscapeFilterOrder=1  InputFilterTimeConstant=0.001  UdotUserProvided=0
      settings: SourceProductBaseCode=SS,PW,VE
  Simulink-PS Converter2 : nesl_utility/Simulink-PS Converter  PhysicalDomain=network_engine_domain  SubClassName=ps_input  LeftPortType=input  RightPortType=output  PseudoPeriodic=off  Frequencies=[]  NoiseDistribution=none  NoiseParameters=[]  Unit=1  AffineConversion=off  FilteringAndDerivatives=provide  SimscapeFilterOrder=1  InputFilterTimeConstant=0.001  UdotUserProvided=0
      settings: SourceProductBaseCode=SS,PW,VE
  To Workspace1 : ToWorkspace  VariableName=qAnkle  SampleTime=-1
  To Workspace2 : ToWorkspace  VariableName=qHip  SampleTime=-1
  To Workspace84 : ToWorkspace  VariableName=qKnee  SampleTime=-1
  excentric branch1 : Fcn  Expr=((5*pi/2) - u) * (u>=(pi/2)) + ((pi/2)-u) *(u<(pi/2))
  left ankle trans : sm_lib/Frames and Transforms/Rigid Transform  TranslationMethod=Cartesian  TranslationStandardOffset=0  TranslationLengthUnit=m  TranslationStandardAxis=+Z  TranslationCartesianOffset=ankle_shank  TranslationROffset=0  TranslationROffsetUnits=m  TranslationZOffset=0  TranslationZOffsetUnits=m  TranslationThetaOffset=0  TranslationThetaOffsetUnits=deg  RotationMethod=StandardAxis  RotationAngleUnits=deg  RotationStandardAxis=+Y  RotationAngle=-90  RotationArbitraryAxis=[0 0 1]  FollAlignAxisA=+X  BaseAlignAxisA=+Y  FollAlignAxisB=+Y  BaseAlignAxisB=+Z  RotationSequenceAxes=FollowerAxes  RotationSequence=XYX  RotationSequenceAngles=[0 0 0]  RotationSequenceAnglesUnits=deg  RotationMatrix=[1 0 0; 0 1 0; 0 0 1]
  left knee trans : sm_lib/Frames and Transforms/Rigid Transform  TranslationMethod=Cartesian  TranslationStandardOffset=0  TranslationLengthUnit=m  TranslationStandardAxis=+Z  TranslationCartesianOffset=knee_thigh * ThPos  TranslationROffset=0  TranslationROffsetUnits=m  TranslationZOffset=0  TranslationZOffsetUnits=m  TranslationThetaOffset=0  TranslationThetaOffsetUnits=deg  RotationMethod=StandardAxis  RotationAngleUnits=deg  RotationStandardAxis=+Y  RotationAngle=-90  RotationArbitraryAxis=[0 0 1]  FollAlignAxisA=+X  BaseAlignAxisA=+Y  FollAlignAxisB=+Y  BaseAlignAxisB=+Z  RotationSequenceAxes=FollowerAxes  RotationSequence=XYX  RotationSequenceAngles=[0 0 0]  RotationSequenceAnglesUnits=deg  RotationMatrix=[1 0 0; 0 1 0; 0 0 1]
  left shank trans : sm_lib/Frames and Transforms/Rigid Transform  TranslationMethod=Cartesian  TranslationStandardOffset=0  TranslationLengthUnit=m  TranslationStandardAxis=+Z  TranslationCartesianOffset=shank_knee  TranslationROffset=0  TranslationROffsetUnits=m  TranslationZOffset=0  TranslationZOffsetUnits=m  TranslationThetaOffset=0  TranslationThetaOffsetUnits=deg  RotationMethod=StandardAxis  RotationAngleUnits=deg  RotationStandardAxis=+Y  RotationAngle=90  RotationArbitraryAxis=[0 0 1]  FollAlignAxisA=+X  BaseAlignAxisA=+Y  FollAlignAxisB=+Y  BaseAlignAxisB=+Z  RotationSequenceAxes=FollowerAxes  RotationSequence=XYX  RotationSequenceAngles=[0 0 0]  RotationSequenceAnglesUnits=deg  RotationMatrix=[1 0 0; 0 1 0; 0 0 1]
  left thigh trans : sm_lib/Frames and Transforms/Rigid Transform  TranslationMethod=Cartesian  TranslationStandardOffset=0  TranslationLengthUnit=m  TranslationStandardAxis=+Z  TranslationCartesianOffset=thigh_hip * (1-ThPos)  TranslationROffset=0  TranslationROffsetUnits=m  TranslationZOffset=0  TranslationZOffsetUnits=m  TranslationThetaOffset=0  TranslationThetaOffsetUnits=deg  RotationMethod=StandardAxis  RotationAngleUnits=deg  RotationStandardAxis=+Y  RotationAngle=90  RotationArbitraryAxis=[0 0 1]  FollAlignAxisA=+X  BaseAlignAxisA=+Y  FollAlignAxisB=+Y  BaseAlignAxisB=+Z  RotationSequenceAxes=FollowerAxes  RotationSequence=XYX  RotationSequenceAngles=[0 0 0]  RotationSequenceAnglesUnits=deg  RotationMatrix=[1 0 0; 0 1 0; 0 0 1]
  map(-pi,pi]to[0,2pi)3 : MATLAB Function  TreatAsAtomicUnit=on
  map(-pi,pi]to[0,2pi)4 : MATLAB Function  TreatAsAtomicUnit=on
  B : PMIOPort  Side=Left
  F : PMIOPort  Port=2  Side=Right
  tag scope: LAnkleBMLMAL=global, LHipBMLMAL=global, LHipState=global, LKneeBMLMAL=global, LKneeState=global, Ldx=global
  wires:
  map(-pi,pi]to[0,2pi)3/1(y) -> To Workspace2/1, Mux/1
  PS-Simulink Converter/1 -> Mux3/1, map(-pi,pi]to[0,2pi)3/1(u)
  PS-Simulink Converter1/1 -> Mux3/2, Gain3/1
  Mux/1 -> [LHipBMLMAL]
  [LhipM] -> Gain/1
  Mux1/1 -> L Knee Joint Sensor/1, [LKneeBMLMAL]
  PS-Simulink Converter2/1 -> map(-pi,pi]to[0,2pi)4/1(u)
  map(-pi,pi]to[0,2pi)4/1(y) -> To Workspace84/1, Mux1/1
  PS-Simulink Converter5/1 -> Gain1/1
  Mux2/1 -> [LAnkleBMLMAL]
  [LankleM] -> Gain2/1
  Gain/1 -> Simulink-PS Converter/1
  [LkneeM] -> Gain4/1
  Gain2/1 -> Simulink-PS Converter2/1
  Gain1/1 -> Mux2/2
  PS-Simulink Converter3/1 -> Mux1/2
  Gain3/1 -> Mux/2
  Left Thigh/1(dx) -> L Thigh Displacement Sensor/1
  L Thigh Displacement Sensor/1 -> [Ldx]
  L Knee Joint Sensor/1 -> [LKneeState]
  Gain4/1 -> Simulink-PS Converter1/1
  PS-Simulink Converter4/1 -> excentric branch1/1
  excentric branch1/1 -> To Workspace1/1, Mux2/1
  Mux3/1 -> [LHipState]
  connections:
  left shank trans/RConn1 -- Left Shank/RConn1 -- left ankle trans/LConn1
  left thigh trans/LConn1 -- Left Hip/RConn1
  Left hip trans/RConn1 -- Left Hip/LConn1
  left shank trans/LConn1 -- Left Knee/RConn1
  Left Knee/LConn1 -- left knee trans/RConn1
  B/RConn1 -- Left hip trans/LConn1
  PS-Simulink Converter/LConn1 -- Left Hip/RConn2
  Simulink-PS Converter/RConn1 -- Left Hip/LConn2
  Simulink-PS Converter2/RConn1 -- Left Ankle/LConn2
  Simulink-PS Converter1/RConn1 -- Left Knee/LConn2
  Left Hip/RConn3 -- PS-Simulink Converter1/LConn1
  PS-Simulink Converter2/LConn1 -- Left Knee/RConn2
  PS-Simulink Converter3/LConn1 -- Left Knee/RConn3
  PS-Simulink Converter4/LConn1 -- Left Ankle/RConn2
  Left Ankle/RConn3 -- PS-Simulink Converter5/LConn1
  left thigh trans/RConn1 -- Left Thigh/LConn1
  Left Thigh/RConn1 -- left knee trans/LConn1
  F/RConn1 -- Left Ankle/RConn1
  left ankle trans/RConn1 -- Left Ankle/LConn1
